simulink library "Yaw_Ideal_Motor_Lib"  (R2025a)
settings: Solver=ode45  StartTime=0.0  StopTime=10.0  RelTol=1e-3  EnableMultiTasking=on
undefined symbols (not defined in the file): WT_Params
libraries: fl_lib x4, nesl_utility x3, sdl_lib x1, Yaw_Gearbox_Lib x1
Description:
  | Copyright 2009-2025 The MathWorks, Inc. MathWorks, Inc.
settings Model: Creator=smiller  LastModifiedBy=smiller
settings SolverCC: AlgebraicLoopSolver=TrustRegion
settings DataIOCC: LimitDataPoints=on  SaveFormat=Array  SignalLoggingSaveFormat=ModelDataLogs  ReturnWorkspaceOutputs=off
settings OptimizationCC: ReuseModelBlockBuffer=off  ExpressionDepthLimit=2147483647.0  LifeSpan=inf
settings DebuggingCC: UnderspecifiedInitializationDetection=Classic  MergeDetectMultiDrivingBlocksExec=none  SolverPrmCheckMsg=warning  FcnCallInpInsideContextMsg=warning  UnconnectedInputMsg=warning  UnconnectedOutputMsg=warning  UnconnectedLineMsg=warning  AllowSymbolicDim=off  StateNameClashWarn=warning  PregeneratedLibrarySubsystemCodeDiagnostic=none  SFUnexpectedBacktrackingDiag=warning  SFNoUnconditionalDefaultTransitionDiag=warning  SFExecutionAtInitializationDiag=none  ArithmeticOperatorsInVariantConditions=warning
settings HardwareCC: ProdBitPerPointer=32.0  ProdBitPerSizeT=32.0  ProdBitPerPtrDiffT=32.0  ProdLargestAtomicFloat=None  ProdIntDivRoundTo=Undefined  ProdEndianess=Unspecified  ProdWordSize=32.0  ProdHWDeviceType=32-bit Generic
settings ModelReferenceCC: EnableRefExpFcnMdlSchedulingChecks=on  PropagateSignalLabelsOutOfModel=off
settings SFSimCC: SimUseLocalCustomCode=off  CustomCodeUndefinedFunction=UseInterfaceOnly
settings RTWCC: RTWUseLocalCustomCode=off  GPUComputeCapability=3.5  DLArmComputeVersion=19.05
settings CodeAppCC: StateflowObjectComments=on
settings GRTTargetCC: TargetLangStandard=C89/C90 (ANSI)  CombineOutputUpdateFcns=off  GRTInterface=on
settings ConfigComp: CovMetricSettings=dw  CovSaveCumulativeToWorkspaceVar=on  CovSaveSingleToWorkspaceVar=on  CovExternalEMLEnable=off  CovSFcnEnable=off

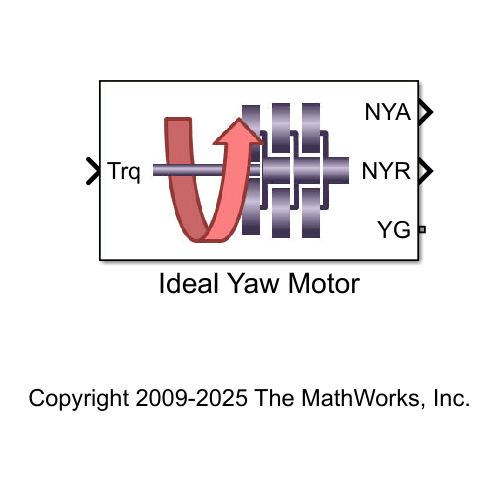
[thumbnail: Simulink's stored preview of the top-level diagram]
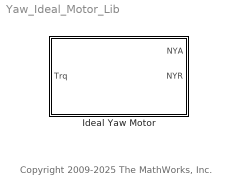
== system Yaw_Ideal_Motor_Lib ==
  note: Copyright 2009-2025 The MathWorks, Inc.
  Ideal Yaw Motor : Subsystem
      mask Display: image('Yaw_Ideal_Motor_Horizontal_IMAGE.jpg');

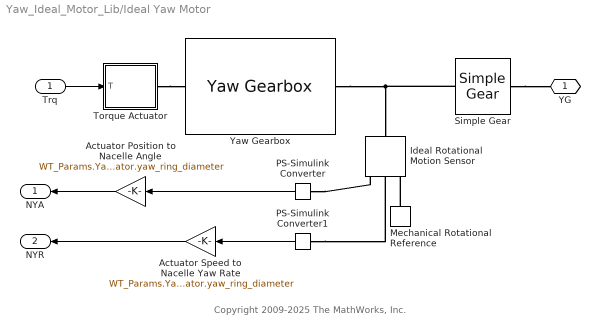
== system Yaw_Ideal_Motor_Lib/Ideal Yaw Motor ==
  note: Copyright 2009-2025 The MathWorks, Inc.
  Trq : Inport
  Actuator Position to Nacelle Angle : Gain  Gain=WT_Params.Yaw_Actuator.yaw_gear_diameter/WT_Params.Yaw_Actuator.yaw_ring_diameter
  Actuator Speed to Nacelle Yaw Rate : Gain  Gain=WT_Params.Yaw_Actuator.yaw_gear_diameter/WT_Params.Yaw_Actuator.yaw_ring_diameter
  Ideal Rotational Motion Sensor : fl_lib/Mechanical/Mechanical Sensors/Ideal Rotational Motion Sensor  reference=foundation.enum.MeasurementReference.difference  acceleration_port=false  velocity_port=true  position_port=true  wrap_angle=simscape.enum.onoff.off  offset=0 rad
  Mechanical Rotational Reference : fl_lib/Mechanical/Rotational Elements/Mechanical Rotational Reference
  PS-Simulink Converter : nesl_utility/PS-Simulink Converter  PhysicalDomain=network_engine_domain  SubClassName=ps_output  LeftPortType=input  RightPortType=output  PseudoPeriodic=off  Frequencies=[]  VectorFormat=1-D array  Unit=deg  AffineConversion=off
  PS-Simulink Converter1 : nesl_utility/PS-Simulink Converter  PhysicalDomain=network_engine_domain  SubClassName=ps_output  LeftPortType=input  RightPortType=output  PseudoPeriodic=off  Frequencies=[]  VectorFormat=1-D array  Unit=deg/s  AffineConversion=off
  Simple Gear : sdl_lib/Gears/Simple Gear  ratio=1/(WT_Params.Yaw_Actuator.yaw_gear_diameter/WT_Params.Yaw_Actuator.yaw_ring_diameter)  rotation_direction=3-2*(2)  friction_model=1  T_noload=0.1 N*m  T_nom=5 N*m  efficiency_nom=0.8  efficiency=0.8  temperature_TLU=[ 280 300 320 ] K  load_TLU=[ 1 5 10 ] N*m  efficiency_TLU=[ 0.95 0.9 0.85 ]  efficiency_TLU2=[ 0.85 0.8 0.75; 0.95 0.9 0.85; 0.85 0.8 0.7 ]  w_thr=0.01 rad/s  pwr_thr=0.001 W  enable_backlash=false  hardstop_model=simscape.enum.hardstop.smooth  backlash_distance=1e-3 mm  r_base=0.1 m  transition=1e-4 mm  backlash_stiffness=1e7 N/m  backlash_damping=1e6 N*s/m  coeff_rest=0  v_tol=0.001 m/s  f_tol=0 N  mu_visc=[ 0 0 ] N*m/(rad/s)  thermal_mass=50 J/K  temperature_specify=off  temperature_priority=High  temperature=300 K  temperature_nominal_specify=off  temperature_nominal_value=1  temperature_nominal_unit=K  x_backlash_specify=off  x_backlash_priority=None  x_backlash=0 mm  x_backlash_nominal_specify=off  x_backlash_nominal_value=1  x_backlash_nominal_unit=mm  f_hardstop_specify=off  f_hardstop_priority=None  f_hardstop=0 N  f_hardstop_nominal_specify=off  f_hardstop_nominal_value=1  f_hardstop_nominal_unit=N  v_backlash_specify=off  v_backlash_priority=None  v_backlash=0 m/s  v_backlash_nominal_specify=off  v_backlash_nominal_value=1  v_backlash_nominal_unit=m/s
  Torque Actuator : Subsystem
      mask Display:
      | plot(400-[198.657636314574;187.5372000791;176.524559560751;165.725772507838;155.244837142898;145.182690602959;135.636236859729;126.697413481378;118.452306223496;110.980319976212;104.353414051689;98.6354091766174;93.8813728637222;90.1370890815176;87.4386173296598;85.811945366254;85.272738931537;85.8261908782356;87.4669711615554;90.1792781704262;93.9369909056548;98.7039205394262;104.434158933498;111.072520759669;118.555074964656;126.809760461083;135.75708011515;145.310866347487;155.379110974044;165.864851295207;176.667103899592;187.681837189509;192.988368326926],[283.691199740558;283.13774779386;281.49696751054;278.784660501669;275.026947766441;270.260018132669;264.529779738597;257.891417912426;250.40886370744;242.154178211013;233.206858556945;223.653072324609;213.584827698051;203.099087376889;192.296834772503;181.282101482586;170.160965409986;159.040529174513;148.027888656163;137.22910160325;126.748166238311;116.686019698372;107.139565955142;98.2007425767901;89.9556353189084;82.4836490716241;75.8567431471018;70.1387382720299;65.3847019591348;61.6404181769301;58.9419464250722;57.3152744616664;56.9214337615639])
      | plot(400-[85.209725657478;1.11807254143059;1.11807254143059], [170.435198815539;170.435198815539;171.380048850551])
      | plot(400-[283.691223012283;397.073227213696], [170.309218810871;170.309218810871])
      | plot(400-[153.301918180659;255.34572196193], [170.309218810871;170.309218810871])
      | plot(400-[198.654719861224;113.618216710165;198.654719861224], [85.2727156598121;170.309218810871;255.34572196193])
      | plot(400-[198.654719861224;153.301918180659;198.654719861224], [215.662020491436;170.309218810871;124.956417130306])
      | plot(400-[198.654719861224;283.691223012283;283.691223012283;187.316519441083;192.985619651154], [283.691223012283;283.691223012283;56.927214609459;56.927214609459;56.927214609459])
      | 
      | patch(400-[395.419739652425;395.419739652425;5.6843418860808e-14;0;395.419739652425;394.947314634919;0.472425017505884;0.472425017505941;394.947314634919;394.947314634919;395.419739652425], [340.618437621742;5.6843418860808e-14;0;340.618437621742;340.618437621742;340.146012604237;340.146012604237;0.472425017505884;0.472425017505884;340.146012604237;340.618437621742], [1;1;1])
      | ;
      | color('red');
      | port_label('RConn', 1,'R')
      | port_label('Input', 1,'T')
  Yaw Gearbox : Yaw_Gearbox_Lib/Yaw Gearbox  SystemSampleTime=-1  VariantActivationTime=update diagram  EmptyChoice=off  PassThrough=off  PassThroughVariantControl=(default)  EmptyChoiceVariantControl=(default)  AllowFlexibleInterface=on  Latency=0  AutoFrameSizeCalculation=off
  YG : PMIOPort  Side=Right
  NYA : Outport  VectorParamsAs1DForOutWhenUnconnected=off
  NYR : Outport  Port=2  VectorParamsAs1DForOutWhenUnconnected=off
  wires:
  PS-Simulink Converter/1 -> Actuator Position to Nacelle Angle/1
  PS-Simulink Converter1/1 -> Actuator Speed to Nacelle Yaw Rate/1
  Actuator Speed to Nacelle Yaw Rate/1 -> NYR/1
  Actuator Position to Nacelle Angle/1 -> NYA/1
  Trq/1 -> Torque Actuator/1(T)
  connections:
  Simple Gear/RConn1 -- YG/RConn1
  Mechanical Rotational Reference/LConn1 -- Ideal Rotational Motion Sensor/RConn1
  PS-Simulink Converter1/LConn1 -- Ideal Rotational Motion Sensor/RConn2
  PS-Simulink Converter/LConn1 -- Ideal Rotational Motion Sensor/RConn3
  Simple Gear/LConn1 -- Ideal Rotational Motion Sensor/LConn1 -- Yaw Gearbox/RConn1
  Torque Actuator/RConn1 -- Yaw Gearbox/LConn1

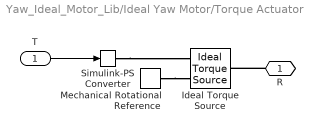
== system Yaw_Ideal_Motor_Lib/Ideal Yaw Motor/Torque Actuator ==
  T : Inport
  Ideal Torque Source : fl_lib/Mechanical/Mechanical Sources/Ideal Torque Source
  Mechanical Rotational Reference : fl_lib/Mechanical/Rotational Elements/Mechanical Rotational Reference
  Simulink-PS Converter : nesl_utility/Simulink-PS Converter  PhysicalDomain=network_engine_domain  SubClassName=ps_input  LeftPortType=input  RightPortType=output  PseudoPeriodic=off  Frequencies=[]  NoiseDistribution=none  NoiseParameters=[]  Unit=1  AffineConversion=off  FilteringAndDerivatives=filter  SimscapeFilterOrder=1  InputFilterTimeConstant=0.005  UdotUserProvided=0
  R : PMIOPort  Side=Right
  wires:
  T/1 -> Simulink-PS Converter/1
  connections:
  R/RConn1 -- Ideal Torque Source/LConn1
  Mechanical Rotational Reference/LConn1 -- Ideal Torque Source/RConn2
  Simulink-PS Converter/RConn1 -- Ideal Torque Source/RConn1
